simulink model "hdlFrame_OpticalFlow_LK_HS_MLFB"  (R2025b)
settings: Solver=FixedStepDiscrete  StopTime=150  EnableMultiTasking=on
InitFcn:
  | thresh=.0015;
  | d5 = [-1 8 0 -8 1]/12;
  | p5 = [1 4 6 4 1]/16;
  | b = ones(1,5)/5;
  | Angle = 98.39185;
  | InitialConditon = 0;
  | line_row = 22;
  | sz = 50;
model workspace (MAT data in the model file):
  SourceMovingObject = 0
  gainValueHSV = 0.2
undefined symbols (not defined in the file or in its folder): gray
libraries: visionconversions x4, visiontextngfix x2, visionsinks x1, dspvision x1
settings Model: Creator=abehbood  LastModifiedBy=jmazur
settings SolverCC: AlgebraicLoopSolver=TrustRegion
settings DataIOCC: ReturnWorkspaceOutputs=off
settings OptimizationCC: ReuseModelBlockBuffer=off  EfficientMapNaN2IntZero=off  LifeSpan=inf
settings DebuggingCC: UnconnectedInputMsg=warning  UnconnectedOutputMsg=warning  UnconnectedLineMsg=warning  SubsystemReferenceDiagnosticForUnitTest=warning  SFUnexpectedBacktrackingDiag=warning  SFNoUnconditionalDefaultTransitionDiag=warning  ArithmeticOperatorsInVariantConditions=warning
settings HardwareCC: TargetBitPerLong=64.0  TargetBitPerPointer=64.0  TargetBitPerSizeT=64.0  TargetBitPerPtrDiffT=64.0  TargetLongLongMode=on  TargetIntDivRoundTo=Zero  TargetEndianess=LittleEndian  TargetWordSize=64.0  TargetHWDeviceType=MATLAB Host  ProdEqTarget=off
settings ModelReferenceCC: EnableRefExpFcnMdlSchedulingChecks=on
settings SFSimCC: SimUseLocalCustomCode=off  CustomCodeUndefinedFunction=UseInterfaceOnly
settings RTWCC: RTWUseLocalCustomCode=off  GPUComputeCapability=3.5  DLArmComputeVersion=19.05
settings CodeAppCC: MaxIdLength=128.0  StateflowObjectComments=on
settings GRTTargetCC: TargetLangStandard=C89/C90 (ANSI)  CombineOutputUpdateFcns=off  GRTInterface=on
settings ConfigComp: CovMetricSettings=dw  CovSaveCumulativeToWorkspaceVar=on  CovSaveSingleToWorkspaceVar=on  CovExternalEMLEnable=off

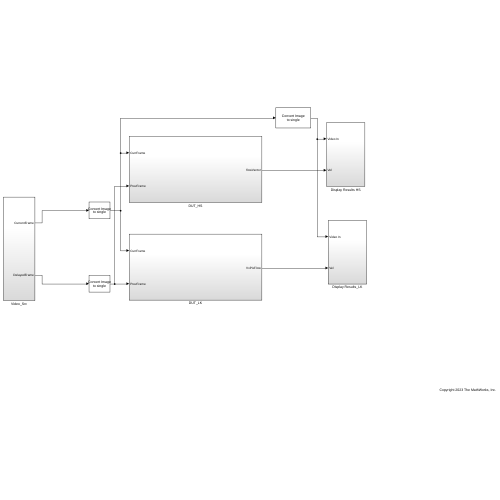
[thumbnail: Simulink's stored preview of the top-level diagram]
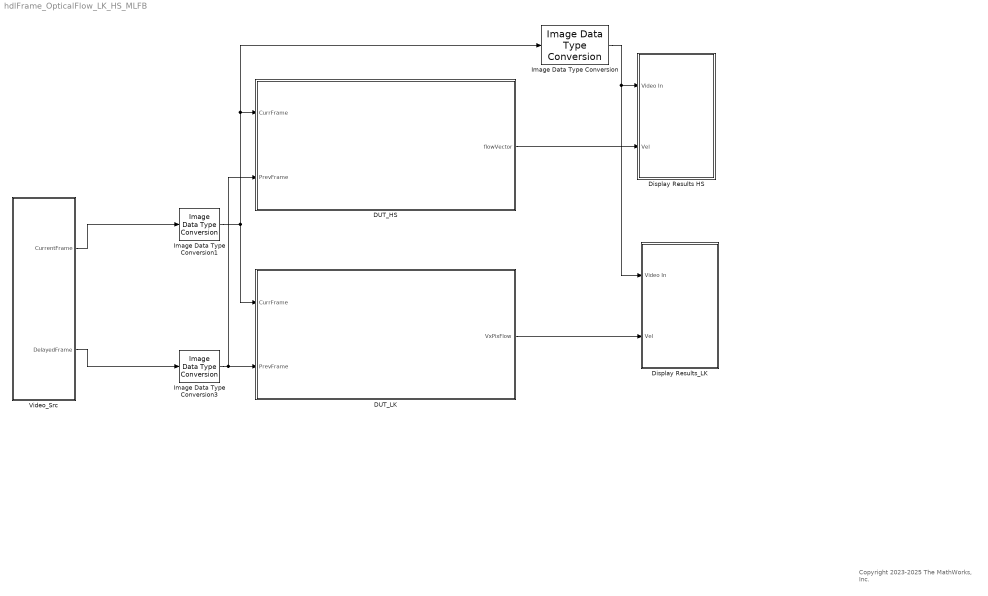
== system hdlFrame_OpticalFlow_LK_HS_MLFB ==
  note: Copyright 2023-2025 The MathWorks, Inc.
  DUT_HS : Subsystem
  DUT_LK : Subsystem
  Display Results HS : Subsystem
  Display Results_LK : Subsystem
  Image Data Type Conversion : visionconversions/Image Data Type Conversion  outDT=single  isSigned=on  wordLen=16  numFracBits=0
  Image Data Type Conversion1 : visionconversions/Image Data Type Conversion  outDT=single  isSigned=on  wordLen=16  numFracBits=0
  Image Data Type Conversion3 : visionconversions/Image Data Type Conversion  outDT=single  isSigned=on  wordLen=16  numFracBits=0
  Video_Src : Subsystem
  wires:
  DUT_HS/1(flowVector) -> Display Results HS/2(Vel)
  Image Data Type Conversion1/1 -> DUT_HS/1(CurrFrame), Image Data Type Conversion/1, DUT_LK/1(CurrFrame)
  Video_Src/2(DelayedFrame) -> Image Data Type Conversion3/1
  DUT_LK/1(VxPixFlow) -> Display Results_LK/2(Vel)
  Video_Src/1(CurrentFrame) -> Image Data Type Conversion1/1
  Image Data Type Conversion/1 -> Display Results_LK/1(Video In), Display Results HS/1(Video In)
  Image Data Type Conversion3/1 -> DUT_LK/2(PrevFrame), DUT_HS/2(PrevFrame)

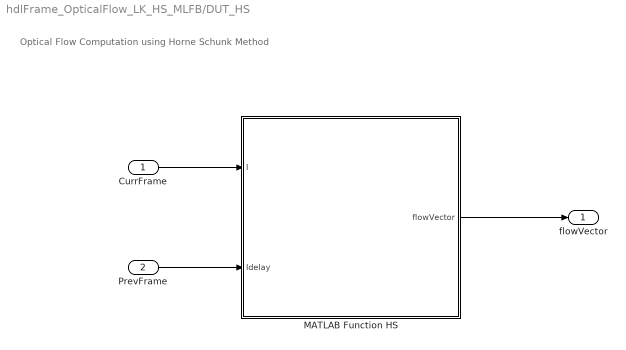
== system hdlFrame_OpticalFlow_LK_HS_MLFB/DUT_HS ==
  note: Optical Flow Computation using Horne Schunk Method
  CurrFrame : Inport
  PrevFrame : Inport  Port=2
  MATLAB Function HS : MATLAB Function  TreatAsAtomicUnit=on
  flowVector : Outport
  wires:
  CurrFrame/1 -> MATLAB Function HS/1(I)
  PrevFrame/1 -> MATLAB Function HS/2(Idelay)
  MATLAB Function HS/1(flowVector) -> flowVector/1

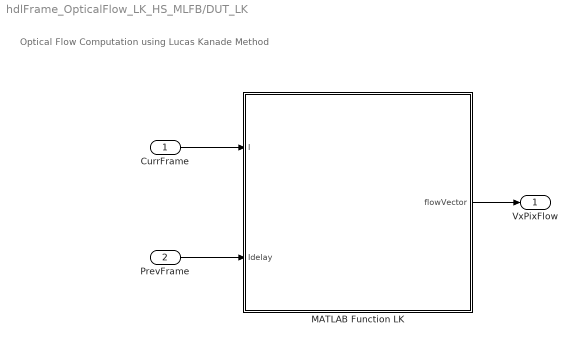
== system hdlFrame_OpticalFlow_LK_HS_MLFB/DUT_LK ==
  note: Optical Flow Computation using Lucas Kanade Method
  CurrFrame : Inport
  PrevFrame : Inport  Port=2
  MATLAB Function LK : MATLAB Function  TreatAsAtomicUnit=on
  VxPixFlow : Outport
  wires:
  PrevFrame/1 -> MATLAB Function LK/2(Idelay)
  CurrFrame/1 -> MATLAB Function LK/1(I)
  MATLAB Function LK/1(flowVector) -> VxPixFlow/1

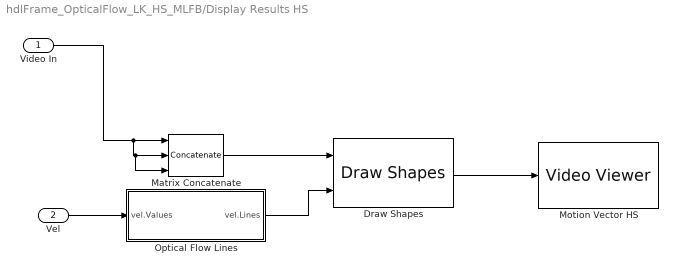
== system hdlFrame_OpticalFlow_LK_HS_MLFB/Display Results HS ==
  Video In : Inport
  Vel : Inport  Port=2
  Draw Shapes : visiontextngfix/Draw Shapes  shape=Lines  fill=off  lineWidth=1  fillClrSource=Specify via dialog  display=User-specified value  intensity=200  color=[255 255 0]  opacity=0.6  viewport=Entire image  antialiasing=off  inType=Obsolete  imagePorts=One multidimensional signal  roundingMode=Floor  overflowMode=off  memoryMode=Specify word length  memoryWordLength=16  prodOutputMode=Binary point scaling  prodOutputWordLength=32  prodOutputFracLength=14  memoryFracLength=15
  Matrix Concatenate : Concatenate  NumInputs=3  Mode=Multidimensional array  ConcatenateDimension=3
  Motion Vector HS : VideoViewer  colormapValue=gray(256)  FigPos=[813 1186 564 350.4]  trueSizedOnce=on
  Optical Flow Lines : Subsystem  mask(Optical Flow Lines){scaleFactor=1}
      mask prompts: scaleFactor "Motion vector gain:"
      mask help: Generates the coordinate points of optical flow lines.
      mask Help: Generates the coordinate points of optical flow lines. Look under its mask to see the implementation details.
  wires:
  Video In/1 -> Matrix Concatenate/3, Matrix Concatenate/2, Matrix Concatenate/1
  Draw Shapes/1 -> Motion Vector HS/1
  Optical Flow Lines/1(vel.Lines) -> Draw Shapes/2
  Vel/1 -> Optical Flow Lines/1(vel.Values)
  Matrix Concatenate/1 -> Draw Shapes/1

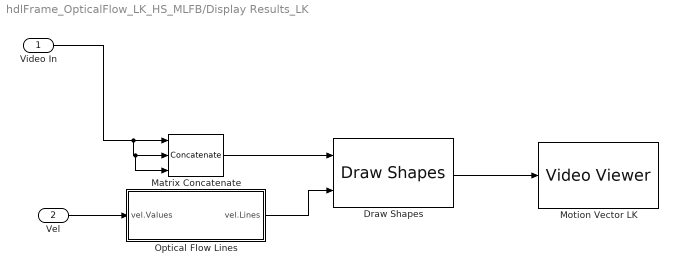
== system hdlFrame_OpticalFlow_LK_HS_MLFB/Display Results_LK ==
  Video In : Inport
  Vel : Inport  Port=2
  Draw Shapes : visiontextngfix/Draw Shapes  shape=Lines  fill=off  lineWidth=1  fillClrSource=Specify via dialog  display=User-specified value  intensity=200  color=[255 255 0]  opacity=0.6  viewport=Entire image  antialiasing=off  inType=Obsolete  imagePorts=One multidimensional signal  roundingMode=Floor  overflowMode=off  memoryMode=Specify word length  memoryWordLength=16  prodOutputMode=Binary point scaling  prodOutputWordLength=32  prodOutputFracLength=14  memoryFracLength=15
  Matrix Concatenate : Concatenate  NumInputs=3  Mode=Multidimensional array  ConcatenateDimension=3
  Motion Vector LK : VideoViewer  colormapValue=gray(256)  FigPos=[1562.33333333333 1185 563.66666666667 350.33333333333]  trueSizedOnce=on
  Optical Flow Lines : Subsystem  mask(Optical Flow Lines){scaleFactor=1}
      mask prompts: scaleFactor "Motion vector gain:"
      mask help: Generates the coordinate points of optical flow lines.
      mask Help: Generates the coordinate points of optical flow lines. Look under its mask to see the implementation details.
  wires:
  Video In/1 -> Matrix Concatenate/3, Matrix Concatenate/2, Matrix Concatenate/1
  Draw Shapes/1 -> Motion Vector LK/1
  Optical Flow Lines/1(vel.Lines) -> Draw Shapes/2
  Vel/1 -> Optical Flow Lines/1(vel.Values)
  Matrix Concatenate/1 -> Draw Shapes/1

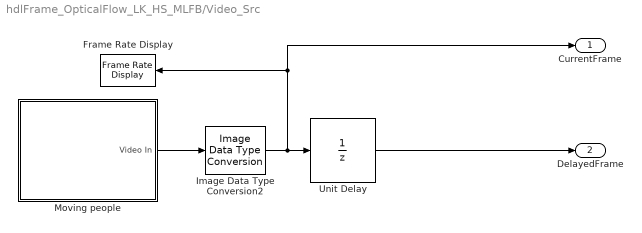
== system hdlFrame_OpticalFlow_LK_HS_MLFB/Video_Src ==
  Frame Rate Display : visionsinks/Frame Rate Display  UpdateRate=10
  Image Data Type Conversion2 : visionconversions/Image Data Type Conversion  outDT=single  isSigned=on  wordLen=16  numFracBits=0
  Moving people : Subsystem
  Unit Delay : UnitDelay  SampleTime=-1
  CurrentFrame : Outport
  DelayedFrame : Outport  Port=2
  wires:
  Moving people/1(Video In) -> Image Data Type Conversion2/1
  Image Data Type Conversion2/1 -> CurrentFrame/1, Frame Rate Display/1, Unit Delay/1
  Unit Delay/1 -> DelayedFrame/1

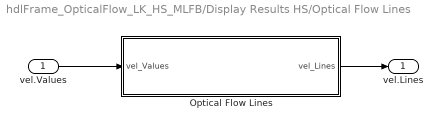
== system hdlFrame_OpticalFlow_LK_HS_MLFB/Display Results HS/Optical Flow Lines ==
  vel.Values : Inport
  Optical Flow Lines : MATLAB Function  TreatAsAtomicUnit=on
  vel.Lines : Outport
  wires:
  Optical Flow Lines/1(vel_Lines) -> vel.Lines/1
  vel.Values/1 -> Optical Flow Lines/1(vel_Values)

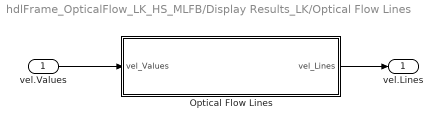
== system hdlFrame_OpticalFlow_LK_HS_MLFB/Display Results_LK/Optical Flow Lines ==
  vel.Values : Inport
  Optical Flow Lines : MATLAB Function  TreatAsAtomicUnit=on
  vel.Lines : Outport
  wires:
  Optical Flow Lines/1(vel_Lines) -> vel.Lines/1
  vel.Values/1 -> Optical Flow Lines/1(vel_Values)

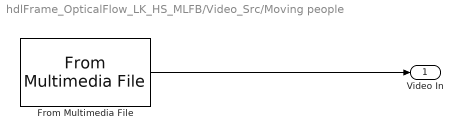
== system hdlFrame_OpticalFlow_LK_HS_MLFB/Video_Src/Moving people ==
  From Multimedia File : dspvision/From Multimedia File  inputFilename=visiontraffic.avi  readRange=[1 Inf]  loop=on  numPlays=inf  outputStreams=Video only  videoDataType=uint8  audioDataType=int16  inheritSampleTime=off  userDefinedSampleTime=1  noAudioOutput=off  isIntensityVideo=off  fourcc=Intensity  colorVideoFormat=One multidimensional signal  outputEOF=off  dataOrg=Column-major  audioFrameSize=1024  computeAudioFrameSize=off  outSamplingMode=Sample based
  Video In : Outport
  wires:
  From Multimedia File/1 -> Video In/1

== matlab function hdlFrame_OpticalFlow_LK_HS_MLFB/Display Results_LK/Optical Flow Lines/Optical Flow Lines ==
  data: vel_Values input; vel_Lines output; scaleFactor parameter size=1
function vel_Lines=OpticalFlowLines(vel_Values, scaleFactor) 

% Generates the coordinate points of optical flow lines

persistent first_time;
persistent X;
persistent Y;
persistent RV;
persistent CV;
if isempty(first_time)
    first_time     = 1;
    %% user may change the following three parameters
    borderOffset   = 5;
    decimFactorRow = 5;
    decimFactorCol = 5;    
    %%
    [R C] = size(vel_Values);
    RV = borderOffset:decimFactorRow:(R-borderOffset);   
    CV = borderOffset:decimFactorCol:(C-borderOffset);
    [Y X] = meshgrid(CV,RV);
end

tmp = vel_Values(RV,CV);
tmp = tmp.*scaleFactor;
vel_Lines = [Y(:), X(:), Y(:)+real(tmp(:)), X(:)+imag(tmp(:))];

== matlab function hdlFrame_OpticalFlow_LK_HS_MLFB/DUT_HS/MATLAB Function HS ==
  data: I input; flowVector output; Idelay input
function flowVector = opticalFlowForHDLBlk(I, Idelay)

flowVector = opticalFlowForHDL_hs(I, Idelay);

end

function [flowVector] = opticalFlowForHDL_hs(I,Id)
%

%   Copyright 2021 The MathWorks, Inc.

%#codegen

%Iterations = 1;
alpha = single(0.99);

%% Brightness Constraints
%Ix = conv2(I, windowFilterHDerivative, 'same');
Ix = hdl.npufun(@imfilter_windowFilterHDerivative, [3 3], I);


%Iy = conv(I, windowFilterVDerivative, 'same');
Iy = hdl.npufun(@imfilter_windowFilterVDerivative, [3 3], I);
It = I - Id;

%v = zeros(size(I));
%u = zeros(size(I));
v = hdl.npufun(@zerosFcn, [1 1], I);
u = hdl.npufun(@zerosFcn, [1 1], I);

%% Smoothness Constrains
%for it = 1:Iterations
    dBrightness = Iy .* v + Ix .* u + It;
    dSmoothness = (Iy .* Iy + Ix .* Ix + alpha * alpha);
    
    vDiff = v - (dBrightness .* Iy ./ dSmoothness);
    %v = conv2(vDiff, windowFilterAveraging, 'same');
    v = hdl.npufun(@imfilter_windowFilterAveraging, [3 3], vDiff);

    
    uDiff = u - (dBrightness .* Ix ./ dSmoothness);
    %u = conv2(uDiff, windowFilterAveraging, 'same');
    u = hdl.npufun(@imfilter_windowFilterAveraging, [3 3], uDiff);    
%end
flowVector = complex(u,v);

end

function z = zerosFcn(I_1x1) %#ok<INUSD>
z = single(0);
end


function WFHD = imfilter_windowFilterHDerivative(I_3x3)

coder.inline('always');
d3x3 = single([-1 -2 -1; 0 0 0; 1 2 1]/8);
windowFilterHDerivative = (d3x3(:));
[WFHD] = sum(windowFilterHDerivative .* I_3x3(:), 'native');


end


function WFHD = imfilter_windowFilterVDerivative(I_3x3)

coder.inline('always');
d3x3 = single([-1 0 1; -2 0 2; -1 0 1]/8);
windowFilterVDerivative = (d3x3(:));
[WFHD] = sum(windowFilterVDerivative .* I_3x3(:), 'native');


end


function WFHD = imfilter_windowFilterAveraging(I_3x3)

coder.inline('always');
d3x3 = single([0 1 0; 1 0 1; 0 1 0]/4);
windowFilterAveraging = (d3x3(:));
[WFHD] = sum(windowFilterAveraging .* I_3x3(:), 'native');


end

== matlab function hdlFrame_OpticalFlow_LK_HS_MLFB/Display Results HS/Optical Flow Lines/Optical Flow Lines ==
  data: vel_Values input; vel_Lines output; scaleFactor parameter size=1
function vel_Lines=OpticalFlowLines(vel_Values, scaleFactor) 

% Generates the coordinate points of optical flow lines

persistent first_time;
persistent X;
persistent Y;
persistent RV;
persistent CV;
if isempty(first_time)
    first_time     = 1;
    %% user may change the following three parameters
    borderOffset   = 5;
    decimFactorRow = 5;
    decimFactorCol = 5;    
    %%
    [R C] = size(vel_Values);
    RV = borderOffset:decimFactorRow:(R-borderOffset);   
    CV = borderOffset:decimFactorCol:(C-borderOffset);
    [Y X] = meshgrid(CV,RV);
end

tmp = vel_Values(RV,CV);
tmp = tmp.*scaleFactor;
vel_Lines = [Y(:), X(:), Y(:)+real(tmp(:)), X(:)+imag(tmp(:))];

== matlab function hdlFrame_OpticalFlow_LK_HS_MLFB/DUT_LK/MATLAB Function LK ==
  data: I input; flowVector output; Idelay input
function flowVector = opticalFlowForHDLBlk(I, Idelay)

flowVector = opticalFlowForHDL_lk(I, Idelay);

end

function [flowVector] = opticalFlowForHDL_lk(I, Idelay)
% Lucas Kanade

%   Copyright 2021 The MathWorks, Inc.

%#codegen

Ix = hdl.npufun(@imfilter_ComputIx, [1 5], I);
Iy = hdl.npufun(@imfilter_ComputIy, [5 1], I);
It = I - Idelay;

WIxx = hdl.npufun(@imfilter_kernel, [5 5], Ix.*Ix);
WIxy = hdl.npufun(@imfilter_kernel, [5 5], Ix.*Iy);
WIyy = hdl.npufun(@imfilter_kernel, [5 5], Iy.*Iy);
WIxt = hdl.npufun(@imfilter_kernel, [5 5], Ix.*It);
WIyt = hdl.npufun(@imfilter_kernel, [5 5], Iy.*It);

[Vx, Vy] = hdl.npufun(@calc_roots_pixel, [1 1], WIxx, WIxy, WIyy, WIxt, WIyt);
flowVector = complex(Vx,Vy);

end

function WI_1x1 = imfilter_ComputIx(I_1x5)

coder.inline('always');

d5 = [-1 8 0 -8 1]/12;
d5 = fliplr(d5(:)');
[WI_1x1] = sum(d5 .* I_1x5);

end

function WI_1x1 = imfilter_ComputIy(I_5x1)

coder.inline('always');

d5 = [-1 8 0 -8 1]/12;
d5 = flipud(d5(:));
[WI_1x1] = sum(d5(:) .* I_5x1);

end

function WI_1x1 = imfilter_kernel(I_5x5)

coder.inline('always');

p5 = [1 4 6 4 1]/16;
W = p5(:)*p5(:)';
[WI_1x1] = sum(W(:) .* I_5x5(:));

end

function [VxPix, VyPix] = calc_roots_pixel(aPix, bPix, cPix, ...
    txPix, tyPix)

coder.inline('always');

r = aPix + cPix;
s = sqrt(single(4 * bPix * bPix + (aPix - cPix) * (aPix - cPix)));
eig1 = (single(r) + s);
eig2 = (single(r) - s);

vx = single(0);
vy = single(0);
% thresh = single(196.6);  %98.3040*2
thresh = 0.0039;
% thresh2 = single(98.304);
thresh2 = 0;

if (eig1 > thresh && eig2 > thresh)
    d = bPix * bPix - aPix * cPix;
    iDelta = 1/d;
    vx =  single( -(tyPix * bPix - txPix * cPix)*iDelta);
    vy =  single( -(txPix * bPix - aPix * tyPix)*iDelta);
elseif (eig1 > thresh && eig2 < thresh)
    rr = bPix+aPix;
    cc = cPix+bPix;
    norm = cc*cc + rr*rr;

    if (norm > thresh2)
        invnorm = 1/norm;
        tmp = -(txPix + tyPix) * invnorm;
        vx =  single(rr * tmp);
        vy =  single(cc * tmp);
    end
end

VxPix = vx;
VyPix = vy;

end
